simulink model "hbridge_rl_verified"  (R2026a)
settings: Solver=FixedStepDiscrete  StartTime=0  StopTime=0.42  FixedStep=1e-6
libraries: ee_lib x14, nesl_utility x8, fl_lib x4
settings Model: ModifiedByFormat=GKC3-Simulink contributors  Creator=GKC3-Simulink contributors  LastModifiedBy=GKC3-Simulink contributors
settings SolverCC: ZeroCrossControl=DisableAll
settings SimscapeCC: EditingMode=Restricted

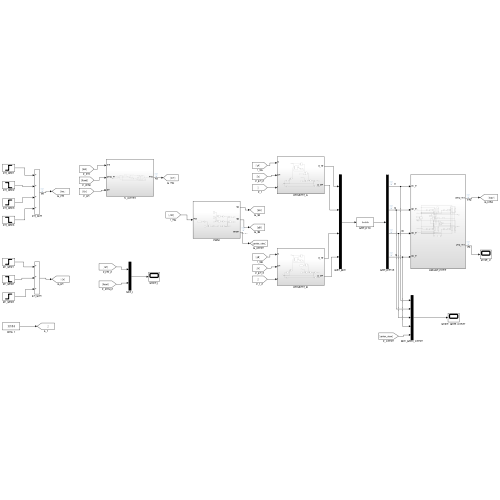
[thumbnail: Simulink's stored preview of the top-level diagram]
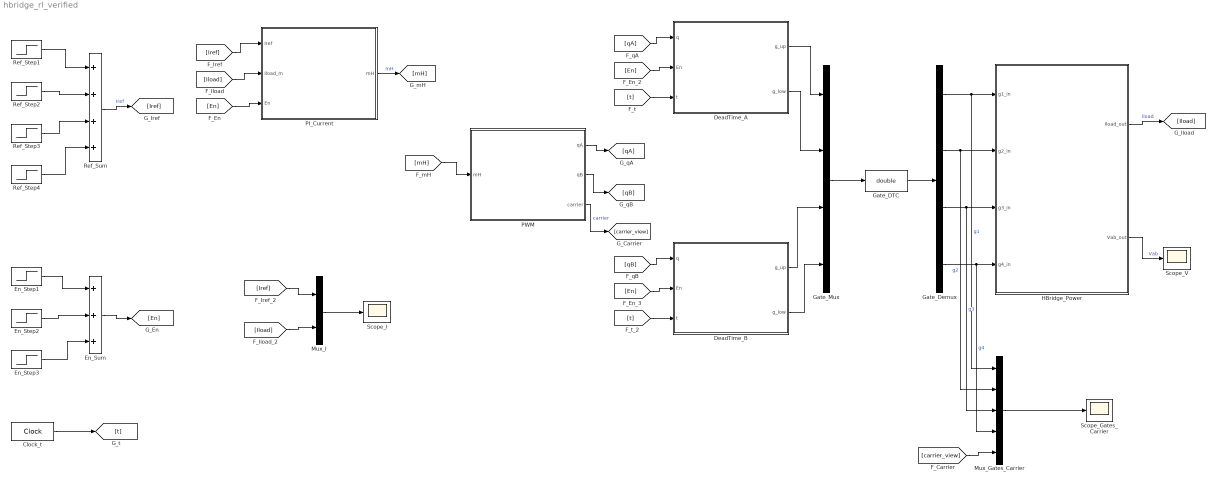
== system hbridge_rl_verified ==
  Clock_t : DigitalClock  SampleTime=1e-6
  DeadTime_A : Subsystem
  DeadTime_B : Subsystem
  En_Step1 : Step  Time=0.002  SampleTime=1e-6
  En_Step2 : Step  Time=0.30  FinalValue=-1  SampleTime=1e-6
  En_Step3 : Step  Time=0.32  SampleTime=1e-6
  En_Sum : Sum  Inputs=+++
  Gate_DTC : DataTypeConversion  OutDataTypeStr=double  SaturateOnIntegerOverflow=off  RndMeth=Floor
  Gate_Demux : Demux
  Gate_Mux : Mux
  HBridge_Power : Subsystem
  Mux_Gates_Carrier : Mux  Inputs=5
  Mux_I : Mux  Inputs=2
  PI_Current : Subsystem
  PWM : Subsystem
  Ref_Step1 : Step  Time=0.02  FinalValue=500  SampleTime=50e-6
  Ref_Step2 : Step  Time=0.12  FinalValue=-1000  SampleTime=50e-6
  Ref_Step3 : Step  Time=0.24  FinalValue=800  SampleTime=50e-6
  Ref_Step4 : Step  Time=0.36  FinalValue=-300  SampleTime=50e-6
  Ref_Sum : Sum  Inputs=++++
  Scope_Gates_Carrier : Scope
  Scope_I : Scope
  Scope_V : Scope
  wires:
  Gate_Mux/1 -> Gate_DTC/1
  DeadTime_B/2(g_low) -> Gate_Mux/4
  DeadTime_B/1(g_up) -> Gate_Mux/3
  DeadTime_A/2(g_low) -> Gate_Mux/2
  DeadTime_A/1(g_up) -> Gate_Mux/1
  [qB] -> DeadTime_B/1(q)
  [qA] -> DeadTime_A/1(q)
  [t] -> DeadTime_B/3(t)
  [t] -> DeadTime_A/3(t)
  Clock_t/1 -> [t]
  [En] -> DeadTime_B/2(En)
  [En] -> DeadTime_A/2(En)
  En_Step2/1 -> En_Sum/2
  En_Step1/1 -> En_Sum/1
  Mux_I/1 -> Scope_I/1
  [Iload] -> Mux_I/2
  [Iref] -> Mux_I/1
  Ref_Sum/1 -> [Iref]  "Iref"
  Ref_Step2/1 -> Ref_Sum/2
  Ref_Step1/1 -> Ref_Sum/1
  Ref_Step3/1 -> Ref_Sum/3
  Ref_Step4/1 -> Ref_Sum/4
  [Iref] -> PI_Current/1(Iref)
  [Iload] -> PI_Current/2(Iload_m)
  En_Step3/1 -> En_Sum/3
  En_Sum/1 -> [En]
  [En] -> PI_Current/3(En)
  PI_Current/1(mH) -> [mH]  "mH"
  Gate_DTC/1 -> Gate_Demux/1
  HBridge_Power/1(Iload_out) -> [Iload]  "Iload"
  HBridge_Power/2(Vab_out) -> Scope_V/1  "Vab"
  Mux_Gates_Carrier/1 -> Scope_Gates_Carrier/1
  Gate_Demux/1 -> Mux_Gates_Carrier/1, HBridge_Power/1(g1_in)  "g1"
  Gate_Demux/2 -> Mux_Gates_Carrier/2, HBridge_Power/2(g2_in)  "g2"
  Gate_Demux/3 -> HBridge_Power/3(g3_in), Mux_Gates_Carrier/3  "g3"
  Gate_Demux/4 -> HBridge_Power/4(g4_in), Mux_Gates_Carrier/4  "g4"
  [carrier_view] -> Mux_Gates_Carrier/5
  PWM/3(carrier) -> [carrier_view]  "carrier"
  [mH] -> PWM/1(mH)
  PWM/1(qA) -> [qA]
  PWM/2(qB) -> [qB]

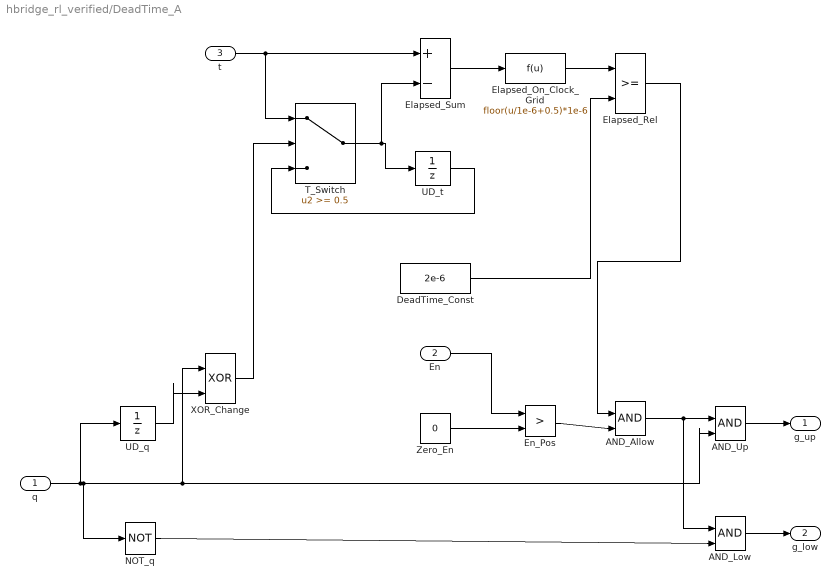
== system hbridge_rl_verified/DeadTime_A ==
  q : Inport
  En : Inport  Port=2
  t : Inport  Port=3
  AND_Allow : Logic  IconShape=distinctive  AllPortsSameDT=off  OutDataTypeStr=boolean
  AND_Low : Logic  IconShape=distinctive  AllPortsSameDT=off  OutDataTypeStr=boolean
  AND_Up : Logic  IconShape=distinctive  AllPortsSameDT=off  OutDataTypeStr=boolean
  DeadTime_Const : Constant  Value=2e-6
  Elapsed_On_Clock_Grid : Fcn  Expr=floor(u/1e-6+0.5)*1e-6
  Elapsed_Rel : RelationalOperator  OutDataTypeStr=boolean  RndMeth=Simplest  InputSameDT=off
  Elapsed_Sum : Sum  Inputs=+-
  En_Pos : RelationalOperator  Operator=>  OutDataTypeStr=boolean  RndMeth=Simplest  InputSameDT=off
  NOT_q : Logic  Operator=NOT  Inputs=1  IconShape=distinctive  AllPortsSameDT=off  OutDataTypeStr=boolean
  T_Switch : Switch  Threshold=0.5  SaturateOnIntegerOverflow=off  InputSameDT=off
  UD_q : UnitDelay  SampleTime=1e-6
  UD_t : UnitDelay  InitialCondition=-1  SampleTime=1e-6
  XOR_Change : Logic  Operator=XOR  IconShape=distinctive  AllPortsSameDT=off  OutDataTypeStr=boolean
  Zero_En : Constant  Value=0
  g_up : Outport
  g_low : Outport  Port=2
  wires:
  AND_Low/1 -> g_low/1
  AND_Up/1 -> g_up/1
  NOT_q/1 -> AND_Low/2
  AND_Allow/1 -> AND_Up/1, AND_Low/1
  En_Pos/1 -> AND_Allow/2
  Zero_En/1 -> En_Pos/2
  En/1 -> En_Pos/1
  T_Switch/1 -> UD_t/1, Elapsed_Sum/2
  UD_t/1 -> T_Switch/3
  XOR_Change/1 -> T_Switch/2
  t/1 -> Elapsed_Sum/1, T_Switch/1
  UD_q/1 -> XOR_Change/2
  q/1 -> AND_Up/2, XOR_Change/1, NOT_q/1, UD_q/1
  Elapsed_On_Clock_Grid/1 -> Elapsed_Rel/1
  Elapsed_Sum/1 -> Elapsed_On_Clock_Grid/1
  DeadTime_Const/1 -> Elapsed_Rel/2
  Elapsed_Rel/1 -> AND_Allow/1

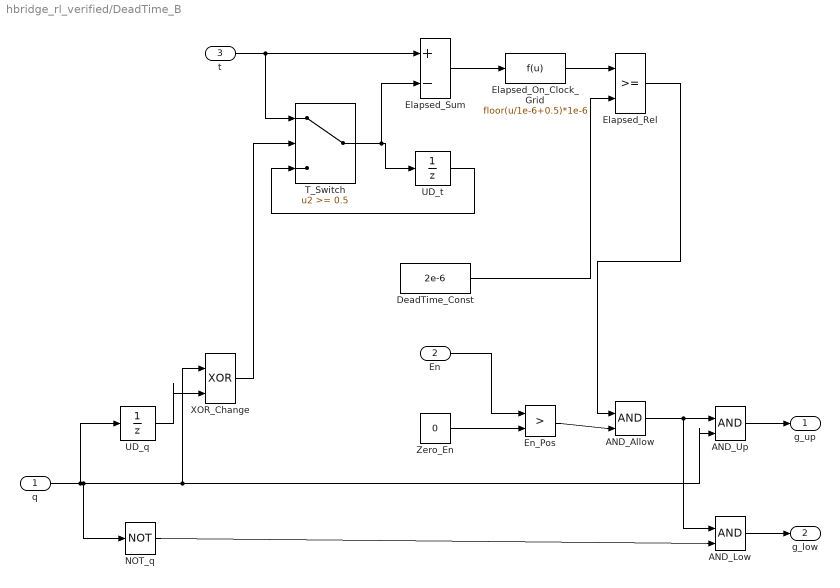
== system hbridge_rl_verified/DeadTime_B ==
  q : Inport
  En : Inport  Port=2
  t : Inport  Port=3
  AND_Allow : Logic  IconShape=distinctive  AllPortsSameDT=off  OutDataTypeStr=boolean
  AND_Low : Logic  IconShape=distinctive  AllPortsSameDT=off  OutDataTypeStr=boolean
  AND_Up : Logic  IconShape=distinctive  AllPortsSameDT=off  OutDataTypeStr=boolean
  DeadTime_Const : Constant  Value=2e-6
  Elapsed_On_Clock_Grid : Fcn  Expr=floor(u/1e-6+0.5)*1e-6
  Elapsed_Rel : RelationalOperator  OutDataTypeStr=boolean  RndMeth=Simplest  InputSameDT=off
  Elapsed_Sum : Sum  Inputs=+-
  En_Pos : RelationalOperator  Operator=>  OutDataTypeStr=boolean  RndMeth=Simplest  InputSameDT=off
  NOT_q : Logic  Operator=NOT  Inputs=1  IconShape=distinctive  AllPortsSameDT=off  OutDataTypeStr=boolean
  T_Switch : Switch  Threshold=0.5  SaturateOnIntegerOverflow=off  InputSameDT=off
  UD_q : UnitDelay  SampleTime=1e-6
  UD_t : UnitDelay  InitialCondition=-1  SampleTime=1e-6
  XOR_Change : Logic  Operator=XOR  IconShape=distinctive  AllPortsSameDT=off  OutDataTypeStr=boolean
  Zero_En : Constant  Value=0
  g_up : Outport
  g_low : Outport  Port=2
  wires:
  AND_Low/1 -> g_low/1
  AND_Up/1 -> g_up/1
  NOT_q/1 -> AND_Low/2
  AND_Allow/1 -> AND_Up/1, AND_Low/1
  En_Pos/1 -> AND_Allow/2
  Zero_En/1 -> En_Pos/2
  En/1 -> En_Pos/1
  T_Switch/1 -> UD_t/1, Elapsed_Sum/2
  UD_t/1 -> T_Switch/3
  XOR_Change/1 -> T_Switch/2
  t/1 -> Elapsed_Sum/1, T_Switch/1
  UD_q/1 -> XOR_Change/2
  q/1 -> AND_Up/2, XOR_Change/1, NOT_q/1, UD_q/1
  Elapsed_On_Clock_Grid/1 -> Elapsed_Rel/1
  Elapsed_Sum/1 -> Elapsed_On_Clock_Grid/1
  DeadTime_Const/1 -> Elapsed_Rel/2
  Elapsed_Rel/1 -> AND_Allow/1

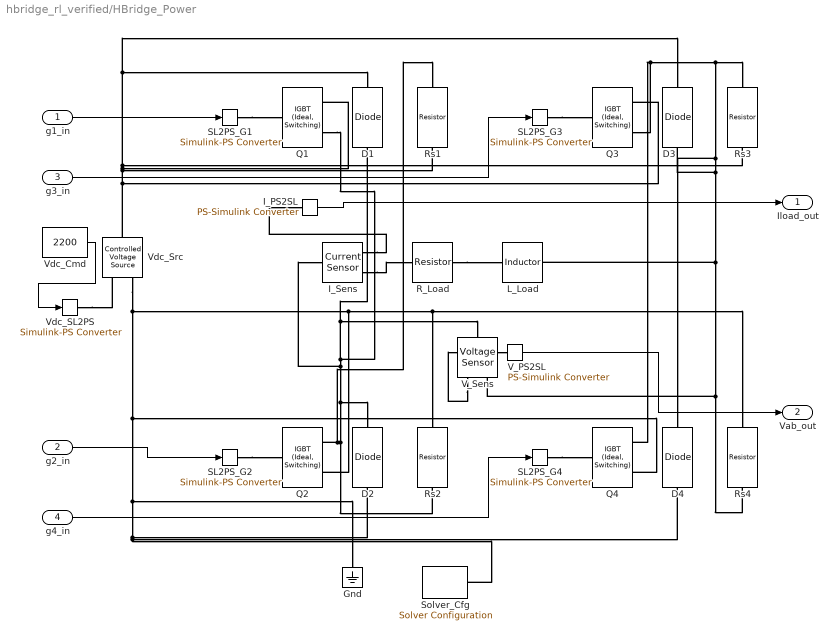
== system hbridge_rl_verified/HBridge_Power ==
  g1_in : Inport
  g2_in : Inport  Port=2
  g3_in : Inport  Port=3
  g4_in : Inport  Port=4
  D{1..4} (4 alike) : ee_lib/Semiconductors & Converters/Diode  ModelType=ee.enum.diode.modelType.pwl  TableType=ee.enum.diode.tableType.IfMat  IfMat=[.07, .12, .19, 1.75, 4.24, 7.32, 11.2; .16, .3, .72, 2.14, 5.02, 8.35, 13.12] A  VfMat=[.9, 1.15, 1.25, 1.5, 1.75, 2.17, 2.6, 2.85; .58, .68, .75, 1.1, 1.38, 1.77, 2.27, 2.7] V  TjVec=[25, 125] degC  VfVec=[.5, .7, .9, 1.3, 1.7, 2.1, 2.5] V  IfVec=[.1, .2, .5, 1, 2, 4, 7, 10] A  IrMat=[1e-06, 2e-06, 5e-06, 1e-05, 2.5e-05, 5e-05, .0001; 2e-06, 5e-06, 1e-05, 4e-05, 8e-05, .0002, .0005] A  VrMat=[10, 100, 200, 250, 300, 325, 350; 10, 70, 160, 220, 270, 300, 320] V  VrVec=[10, 20, 40, 50, 70, 80, 100] V  IrVec=[1e-06, 2e-06, 5e-06, 1e-05, 2e-05, 5e-05, .0001] A  Vf=2 V  Ron=20e-6 Ohm  Goff=1e-8 S  prmExp=ee.enum.diode.expParam.useTwo  I12=[.0137, .545] A  V12=[.6, .7] V  RS=0 Ohm  Tmeas=298.15 K  IS=1e-12 A  ec=1  I1=0.0137 A  V1=0.6 V  N_series=1  N_parallel=1  ZenerEnable=false  Rz=0.3 Ohm  BV=30 V  C_param=ee.enum.diode.capParam.fixed  CJ=0 pF  CJ0=5 pF  Vvec=[.1, 10, 100] V  Cvec=[3.5, 1, .4] pF  VJ=1 V  Mgrad=0.5  FC=0.5  Q_param=ee.enum.diode.recoveryParam.off  iRM=-7.15 A  iF=4 A  didt=-750 A/us  trr_factor=3  trr=115 ns  Qrr=150 nA*s  Vr=-600 V  Ls=150 nH  Erec=0.03 J  TT=50 ns  tau=100 ns  T_param=ee.enum.diode.temperatureParam.off  Tdevice=298.15 K  I1_T2=0.245 A  V1_T2=0.5 V  IS_T2=1.25e-7 A  Tmeas2=125 degC  XTI_param=ee.enum.diode.xtiParam.pn  XTI=3  EG_param=ee.enum.diode.egapParam.material_si  EG=1.11 eV  dBVdT=0 V/K  enable_fault_input=simscape.enum.onoff.off  i_specify=off  i_priority=None  i=0 A  i_nominal_specify=off  i_nominal_value=1  i_nominal_unit=A  v_specify=off  v_priority=None  v=0 V  v_nominal_specify=off  v_nominal_value=1  v_nominal_unit=V  v_capacitor_specify=off  v_capacitor_priority=None  v_capacitor=0 V  v_capacitor_nominal_specify=off  v_capacitor_nominal_value=1  v_capacitor_nominal_unit=V  Qj_specify=off  Qj_priority=High  Qj=0 C  Qj_nominal_specify=off  Qj_nominal_value=1  Qj_nominal_unit=C  i_diode_specify=off  i_diode_priority=None  i_diode=0 A  i_diode_nominal_specify=off  i_diode_nominal_value=1  i_diode_nominal_unit=A  v_diode_specify=off  v_diode_priority=None  v_diode=0 V  v_diode_nominal_specify=off  v_diode_nominal_value=1  v_diode_nominal_unit=V  i_capacitor_specify=off  i_capacitor_priority=None  i_capacitor=0 A  i_capacitor_nominal_specify=off  i_capacitor_nominal_value=1  i_capacitor_nominal_unit=A  fidelity_level=ee.enum.diode.fidelity.includeChargeDyn  rec_loss_model=ee.enum.diode.reverseRecoveryModelTabulateUpTo3D.fixed  ErecVal=0 J  scaleWithIandV=true  ErecMat=zeros(2, 3) J  ErecMat3D=zeros(2, 3, 2) J  TjrecVec=[298.15, 398.15] K  IfrecVec=[.1, 1, 10] A  IrecVal=10 A  VrecVal=10 V  VrecVec=[0, 100] V  tFilter=1 / 1000 / 100 s  thermal_network_parameterization=ee.enum.thermalNetworkTopology.junctionCase  Rth=[0, 10] K/W  Rth_Cauer=[1, 3, 10] K/W  Rth_Foster=[.08, .14, .22, .16] K/W  thermal_mass_parameterization=ee.enum.thermalNetwork.timeconstant  thermal_mass=[0, 1] J/K  thermal_mass_Cauer=[.1, .3, 1] J/K  thermal_mass_Foster=[.001, .005, .05, .5] J/K  thermal_time_constant=[0, 10] s  thermal_time_constant_Cauer=[1, 3, 10] s  thermal_time_constant_Foster=[7e-05, .0007, .01, .08] s  thermal_mass_initial_temperatures=[25, 25] degC  thermal_mass_initial_temperatures_Cauer=[25, 25, 25] degC  junction_thermal_mass=0.01 J/K  Tvec_initial_Foster=[25, 25, 25, 25] degC  no_thermal_network=0  junction_temperature_specify=off  junction_temperature_priority=None  junction_temperature=25 degC  junction_temperature_nominal_specify=off  junction_temperature_nominal_value=1  junction_temperature_nominal_unit=degC
  Gnd : fl_lib/Electrical/Electrical Elements/Electrical Reference
  I_PS2SL : nesl_utility/PS-Simulink Converter  PhysicalDomain=network_engine_domain  SubClassName=ps_output  LeftPortType=input  RightPortType=output  PseudoPeriodic=off  Frequencies=[]  VectorFormat=inherit  Unit=A  AffineConversion=off
  I_Sens : fl_lib/Electrical/Electrical Sensors/Current Sensor
  L_Load : ee_lib/Passive/Inductor  l=20e-3 H  enable_L_tol=ee.enum.toleranceApplication.none  L_tol=20  tol_distribution=ee.enum.toleranceDistribution.uniform  nSigma=4  r=0 Ohm  g=0 1/Ohm  enable_operating_limits=ee.enum.enable.no  operating_limit_action=ee.enum.passive.reportOpLim.warn  max_working_current=1 A  power_rating=1 W  i_L_specify=on  i_L_priority=High  i_L=0 A  i_L_nominal_specify=off  i_L_nominal_value=1  i_L_nominal_unit=A
  Q{1..4} (4 alike) : ee_lib/Semiconductors & Converters/IGBT (Ideal, Switching)  port_option=ee.enum.controlport.ps  Vf=2 V  Ron=20e-6 Ohm  Goff=1e-8 1/Ohm  Vth=0.5 V  diode_param=ee.enum.semiconductors.protectionDiode.external  diode_Vf=0.8 V  diode_Ron=0.001 Ohm  diode_Goff=1e-5 1/Ohm  diode_C=50e-9 F  diode_iRM=-235 A  diode_iF=300 A  diode_idot=-50 A/us  diode_trr_param=ee.enum.converters.diodeReverseParam.trr_factor  diode_trr_factor=3  diode_trr=15 us  diode_Qrr=1500 s*uA  ice_specify=off  ice_priority=None  ice=0 A  ice_nominal_specify=off  ice_nominal_value=1  ice_nominal_unit=A  vce_specify=off  vce_priority=None  vce=0 V  vce_nominal_specify=off  vce_nominal_value=1  vce_nominal_unit=V  vge_specify=off  vge_priority=None  vge=0 V  vge_nominal_specify=off  vge_nominal_value=1  vge_nominal_unit=V  thermal_loss_option=ee.enum.converters.thermalLossOption.constantvalues  Von_data=[0, .1, .6, .8, 1, 1.3, 1.6, 2, 2.4; 0, .1, .7, 1, 1.2, 1.5, 1.9, 2.4, 2.8] V  Tj=[298.15, 398.15] K  Iout_data=[0, .1, 1, 5, 10, 20, 40, 70, 100] A  tabulateWithVce=false  Eon_data=[0, .0024, .024, .12, .2, .48, 1.04, 2.16, 3.24; 0, .003, .03, .15, .25, .6, 1.3, 2.7, 4.05] * 1e-3 J  Eoff_data=[0, .0007, .0066, .033, .066, .17, .33, .83, 1.5; 0, .001, .01, .05, .1, .25, .5, 1.2, 2.2] * 1e-3 J  Eon_data_3D=[zeros(2, 9, 3)] J  Eoff_data_3D=[zeros(2, 9, 3)] J  Tj_loss=[298.15, 398.15] K  Iout_data_loss=[0, .1, 1, 5, 10, 20, 40, 70, 100] A  Vce_loss=[0, 150, 300] V  Eon_scalar=22.86e-3 J  Eoff_scalar=17.14e-3 J  Voff=300 V  Iout_scalar=600 A  useCurrentFromPreviousCycle=false  useVoltageFromPreviousCycle=false  diodeModelType=ee.enum.converters.diodeModelType.pwl  diodeTableType=ee.enum.diode.tableType.IfMat  diode_ReverseIVType=ee.enum.diode.diodeReverseIV.constant  diode_IfMat=[.07, .12, .19, 1.75, 4.24, 7.32, 11.2; .16, .3, .72, 2.14, 4.02, 6.35, 9.12] A  diode_VfMat=[.9, 1.15, 1.25, 1.5, 1.75, 2.17, 2.6, 2.85; .58, .68, .75, 1.1, 1.38, 1.77, 2.27, 2.7] V  diode_TjVec=[25, 125] degC  diode_VfVec=[.5, .7, .9, 1.3, 1.7, 2.1, 2.5] V  diode_IfVec=[.1, .2, .5, 1, 2, 4, 7, 10] A  diode_IrMat=[1e-06, 2e-06, 5e-06, 1e-05, 2.5e-05, 5e-05, .0001; 2e-06, 5e-06, 1e-05, 4e-05, 8e-05, .0002, .0005] A  diode_VrMat=[10, 100, 200, 250, 300, 325, 350; 10, 70, 160, 220, 270, 300, 320] V  diode_VrVec=[10, 20, 40, 50, 70, 80, 100] V  diode_IrVec=[1e-06, 2e-06, 5e-06, 1e-05, 2e-05, 5e-05, .0001] A  diode_Vr=-600 V  diode_Ls=150 nH  diode_Erec=0.03 J  diode_rec_loss_model=ee.enum.diode.reverseRecoveryModelTabulateUpTo3D.fixed  diode_ErecVal=0 J  diode_scaleWithIandV=true  diode_ErecMat=zeros(2, 3) J  diodeErecMat3D=zeros(2, 3, 2) J  diode_TjrecVec=[298.15, 398.15] K  diode_IfrecVec=[.1, 1, 10] A  diodeVrecVec=[0, 100] V  diode_IrecVal=10 A  diode_VrecVal=10 V  diode_tFilter=1 / 1000 / 100 s  separateThermalPortForDiode=false  thermal_network_parameterization=ee.enum.thermalNetworkTopology.external  Rth=[.08, .5] K/W  Rth_Cauer=[.08, .1, .5] K/W  Rth_Foster=[.08, .14, .22, .16] K/W  thermal_mass_parameterization=ee.enum.thermalNetwork.timeconstant  thermal_mass=[.01, .5] J/K  thermal_mass_Cauer=[.01, .1, .5] J/K  thermal_mass_Foster=[.001, .005, .05, .5] J/K  thermal_time_constant=[.001, .2] s  thermal_time_constant_Cauer=[.001, .1, .2] s  thermal_time_constant_Foster=[7e-05, .0007, .01, .08] s  thermal_mass_initial_temperatures=[25, 25] degC  thermal_mass_initial_temperatures_Cauer=[25, 25, 25] degC  junction_thermal_mass=0.01 J/K  Tvec_initial_Foster=[25, 25, 25, 25] degC  RthDiode=[.03, .2] K/W  RthCauerDiode=[.03, .1, .2] K/W  RthFosterDiode=[.03, .2] K/W  thermalMassDiode=[3, 25] J/K  thermalMassCauerDiode=[3, 10, 25] J/K  thermalMassFosterDiode=[33, 50] J/K  thermalTauDiode=[.1, 5] s  thermalTauCauerDiode=[.1, 1, 5] s  thermalTauFosterDiode=[1, 10] s  thermalMassInitTempDiode=[25, 25] degC  thermalMassInitTempCauerDiode=[25, 25, 25] degC  junctionthermalMassDiode=0.1 J/K  TVecInitialFosterDiode=[25, 25, 25, 25] degC  no_thermal_network=ee.enum.enable.no  IGBT_junction_temperature_specify=off  IGBT_junction_temperature_priority=None  IGBT_junction_temperature=25 degC  IGBT_junction_temperature_nominal_specify=off  IGBT_junction_temperature_nominal_value=1  IGBT_junction_temperature_nominal_unit=degC  diode_junction_temperature_specify=off  diode_junction_temperature_priority=None  diode_junction_temperature=25 degC  diode_junction_temperature_nominal_specify=off  diode_junction_temperature_nominal_value=1  diode_junction_temperature_nominal_unit=degC  Qj_specify=off  Qj_priority=None  Qj=0 W  Qj_nominal_specify=off  Qj_nominal_value=1  Qj_nominal_unit=W  accumulatedSwitchingLosses_specify=off  accumulatedSwitchingLosses_priority=None  accumulatedSwitchingLosses=0 J
  R_Load : ee_lib/Passive/Resistor  R=0.2 Ohm  enable_R_tol=ee.enum.toleranceApplication.none  R_tol=5  tol_distribution=ee.enum.toleranceDistribution.uniform  nSigma=4  enable_operating_limits=ee.enum.enable.no  operating_limit_action=ee.enum.passive.reportOpLim.warn  power_rating=1 W  max_working_voltage=100 V  noise_mode=ee.enum.sources.noise.Disabled  Tdevice=25 degC  sample_time=1e-3 s  repeatability=ee.enum.ic.repeatability.notRepeatable  user_seed=0  auto_seed=1913778160  power_derating_T1=70 degC  power_derating_T2=155 degC  operating_temperature_range_vec=[-50, 150] degC  alpha=3.93e-3 1/K  Tmeas=25 degC  thermal_mass=100 J/K  temperature_specify=off  temperature_priority=High  temperature=298.15 K  temperature_nominal_specify=off  temperature_nominal_value=1  temperature_nominal_unit=K
  Rs1 : ee_lib/Passive/Resistor  R=1e7 Ohm  enable_R_tol=ee.enum.toleranceApplication.none  R_tol=5  tol_distribution=ee.enum.toleranceDistribution.uniform  nSigma=4  enable_operating_limits=ee.enum.enable.no  operating_limit_action=ee.enum.passive.reportOpLim.warn  power_rating=1 W  max_working_voltage=100 V  noise_mode=ee.enum.sources.noise.Disabled  Tdevice=25 degC  sample_time=1e-3 s  repeatability=ee.enum.ic.repeatability.notRepeatable  user_seed=0  auto_seed=3287869569  power_derating_T1=70 degC  power_derating_T2=155 degC  operating_temperature_range_vec=[-50, 150] degC  alpha=3.93e-3 1/K  Tmeas=25 degC  thermal_mass=100 J/K  temperature_specify=off  temperature_priority=High  temperature=298.15 K  temperature_nominal_specify=off  temperature_nominal_value=1  temperature_nominal_unit=K
  Rs2 : ee_lib/Passive/Resistor  R=1e7 Ohm  enable_R_tol=ee.enum.toleranceApplication.none  R_tol=5  tol_distribution=ee.enum.toleranceDistribution.uniform  nSigma=4  enable_operating_limits=ee.enum.enable.no  operating_limit_action=ee.enum.passive.reportOpLim.warn  power_rating=1 W  max_working_voltage=100 V  noise_mode=ee.enum.sources.noise.Disabled  Tdevice=25 degC  sample_time=1e-3 s  repeatability=ee.enum.ic.repeatability.notRepeatable  user_seed=0  auto_seed=3415357569  power_derating_T1=70 degC  power_derating_T2=155 degC  operating_temperature_range_vec=[-50, 150] degC  alpha=3.93e-3 1/K  Tmeas=25 degC  thermal_mass=100 J/K  temperature_specify=off  temperature_priority=High  temperature=298.15 K  temperature_nominal_specify=off  temperature_nominal_value=1  temperature_nominal_unit=K
  Rs3 : ee_lib/Passive/Resistor  R=1e7 Ohm  enable_R_tol=ee.enum.toleranceApplication.none  R_tol=5  tol_distribution=ee.enum.toleranceDistribution.uniform  nSigma=4  enable_operating_limits=ee.enum.enable.no  operating_limit_action=ee.enum.passive.reportOpLim.warn  power_rating=1 W  max_working_voltage=100 V  noise_mode=ee.enum.sources.noise.Disabled  Tdevice=25 degC  sample_time=1e-3 s  repeatability=ee.enum.ic.repeatability.notRepeatable  user_seed=0  auto_seed=802611725  power_derating_T1=70 degC  power_derating_T2=155 degC  operating_temperature_range_vec=[-50, 150] degC  alpha=3.93e-3 1/K  Tmeas=25 degC  thermal_mass=100 J/K  temperature_specify=off  temperature_priority=High  temperature=298.15 K  temperature_nominal_specify=off  temperature_nominal_value=1  temperature_nominal_unit=K
  Rs4 : ee_lib/Passive/Resistor  R=1e7 Ohm  enable_R_tol=ee.enum.toleranceApplication.none  R_tol=5  tol_distribution=ee.enum.toleranceDistribution.uniform  nSigma=4  enable_operating_limits=ee.enum.enable.no  operating_limit_action=ee.enum.passive.reportOpLim.warn  power_rating=1 W  max_working_voltage=100 V  noise_mode=ee.enum.sources.noise.Disabled  Tdevice=25 degC  sample_time=1e-3 s  repeatability=ee.enum.ic.repeatability.notRepeatable  user_seed=0  auto_seed=2103522063  power_derating_T1=70 degC  power_derating_T2=155 degC  operating_temperature_range_vec=[-50, 150] degC  alpha=3.93e-3 1/K  Tmeas=25 degC  thermal_mass=100 J/K  temperature_specify=off  temperature_priority=High  temperature=298.15 K  temperature_nominal_specify=off  temperature_nominal_value=1  temperature_nominal_unit=K
  SL2PS_G{1..4} (4 alike) : nesl_utility/Simulink-PS Converter  PhysicalDomain=network_engine_domain  SubClassName=ps_input  LeftPortType=input  RightPortType=output  PseudoPeriodic=off  Frequencies=[]  NoiseDistribution=none  NoiseParameters=[]  Unit=V  AffineConversion=off  FilteringAndDerivatives=zero  SimscapeFilterOrder=1  InputFilterTimeConstant=0.001  UdotUserProvided=0
  Solver_Cfg : nesl_utility/Solver Configuration  PhysicalDomain=network_engine_domain  SubClassName=solver  LeftPortType=input  RightPortType=generic  Tones=[]  Harmonics=[]  SimulateNoise=off  Profile=off  UseLocalSampling=off  EnableSwitchedLinearOptims=on  FrequencyDomain=off  UseCCode=off  RelTol=0.001  AbsTol=0.001  MinStep=1e-09  ToWorkspace=off  RevertToSquareIcSolve=off  NumHomotopyIterations=100  PhasorMode=off  PhasorModeNumHarmonics=1  ConsistencySolver=NEWTON_XTOL_AFTER_FTOL  CanonicalOrdering=CANONICAL  OptimizeIntermediates=OPTIMIZED  IndexReductionMethod=DerivativeReplacement  DoDC=off  ResidualTolerance=1e-09  ConsistencyTolSource=GLOBAL  ConsistencyAbsTol=0.001  ConsistencyRelTol=0.001  ConsistencyTolFactor=0.001  UseLocalSolver=on  LocalSolverChoice=NE_BACKWARD_EULER_ADVANCER  ResolveIndetEquations=on  FunctionEvalNumThread=1  LocalSolverSampleTime=1e-6  DoFixedCost=on  MaxNonlinIter=3  MaxModeIter=2  ComputeImpulses=off  ImpulseIterations=2  LinearAlgebra=auto  LinearAlgebraNumThread=0  EquationFormulation=NE_TIME_EF  DelaysMemoryBudget=1024  AutomaticFiltering=on  FilteringTimeConstant=0.001  PartitionStorageMethod=AS_NEEDED  PartitionMemoryBudget=1024  PartitionMethod=ROBUST  MultibodyUseLocalSolver=off  MultibodyLocalSolverChoice=ODE1  MultibodyLocalSolverSampleTime=0.001
  V_PS2SL : nesl_utility/PS-Simulink Converter  PhysicalDomain=network_engine_domain  SubClassName=ps_output  LeftPortType=input  RightPortType=output  PseudoPeriodic=off  Frequencies=[]  VectorFormat=inherit  Unit=V  AffineConversion=off
  V_Sens : fl_lib/Electrical/Electrical Sensors/Voltage Sensor
  Vdc_Cmd : Constant  Value=2200
  Vdc_SL2PS : nesl_utility/Simulink-PS Converter  PhysicalDomain=network_engine_domain  SubClassName=ps_input  LeftPortType=input  RightPortType=output  PseudoPeriodic=off  Frequencies=[]  NoiseDistribution=none  NoiseParameters=[]  Unit=V  AffineConversion=off  FilteringAndDerivatives=zero  SimscapeFilterOrder=1  InputFilterTimeConstant=0.001  UdotUserProvided=0
  Vdc_Src : fl_lib/Electrical/Electrical Sources/Controlled Voltage Source
  Iload_out : Outport
  Vab_out : Outport  Port=2
  wires:
  Vdc_Cmd/1 -> Vdc_SL2PS/1
  V_PS2SL/1 -> Vab_out/1
  I_PS2SL/1 -> Iload_out/1
  g4_in/1 -> SL2PS_G4/1
  g3_in/1 -> SL2PS_G3/1
  g2_in/1 -> SL2PS_G2/1
  g1_in/1 -> SL2PS_G1/1
  connections:
  V_Sens/RConn1 -- V_PS2SL/LConn1
  I_Sens/RConn1 -- I_PS2SL/LConn1
  SL2PS_G4/RConn1 -- Q4/LConn1
  SL2PS_G3/RConn1 -- Q3/LConn1
  SL2PS_G2/RConn1 -- Q2/LConn1
  SL2PS_G1/RConn1 -- Q1/LConn1
  Vdc_SL2PS/RConn1 -- Vdc_Src/RConn1
  R_Load/RConn1 -- L_Load/LConn1
  I_Sens/RConn2 -- R_Load/LConn1
  Q4/RConn1 -- V_Sens/RConn2 -- Rs4/LConn1 -- L_Load/RConn1 -- D3/LConn1 -- D4/RConn1 -- Rs3/RConn1 -- Q3/RConn2
  V_Sens/LConn1 -- Q2/RConn1 -- Rs1/RConn1 -- Rs2/LConn1 -- D2/RConn1 -- I_Sens/LConn1 -- Q1/RConn2 -- D1/LConn1
  Solver_Cfg/RConn1 -- Vdc_Src/RConn2 -- Rs4/RConn1 -- Rs2/RConn1 -- Q2/RConn2 -- Q4/RConn2 -- Gnd/LConn1 -- D2/LConn1 -- D4/LConn1
  Q1/RConn1 -- D1/RConn1 -- D3/RConn1 -- Rs3/LConn1 -- Vdc_Src/LConn1 -- Q3/RConn1 -- Rs1/LConn1

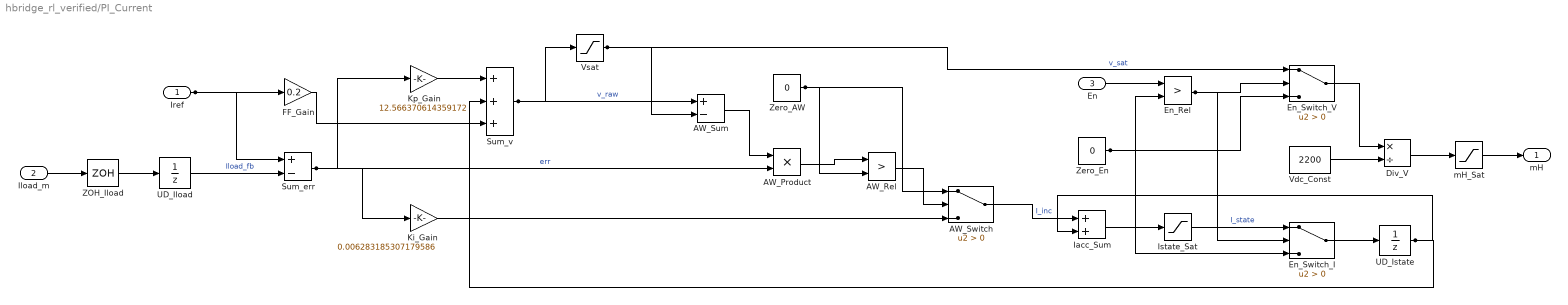
== system hbridge_rl_verified/PI_Current ==
  Iref : Inport
  Iload_m : Inport  Port=2
  En : Inport  Port=3
  AW_Product : Product
  AW_Rel : RelationalOperator  Operator=>  OutDataTypeStr=boolean  RndMeth=Simplest  InputSameDT=off
  AW_Sum : Sum  Inputs=+-
  AW_Switch : Switch  Criteria=u2 > Threshold  SaturateOnIntegerOverflow=off  InputSameDT=off
  Div_V : Product  Inputs=*/
  En_Rel : RelationalOperator  Operator=>  OutDataTypeStr=boolean  RndMeth=Simplest  InputSameDT=off
  En_Switch_I : Switch  Criteria=u2 > Threshold  SaturateOnIntegerOverflow=off  InputSameDT=off
  En_Switch_V : Switch  Criteria=u2 > Threshold  SaturateOnIntegerOverflow=off  InputSameDT=off
  FF_Gain : Gain  Gain=0.2
  Iacc_Sum : Sum
  Istate_Sat : Saturate  UpperLimit=400  LowerLimit=-400
  Ki_Gain : Gain  Gain=0.006283185307179586
  Kp_Gain : Gain  Gain=12.566370614359172
  Sum_err : Sum  Inputs=+-
  Sum_v : Sum  Inputs=+++
  UD_Iload : UnitDelay  SampleTime=50e-6
  UD_Istate : UnitDelay  SampleTime=50e-6
  Vdc_Const : Constant  Value=2200
  Vsat : Saturate  UpperLimit=400  LowerLimit=-400
  ZOH_Iload : ZeroOrderHold  SampleTime=50e-6
  Zero_AW : Constant  Value=0
  Zero_En : Constant  Value=0
  mH_Sat : Saturate  UpperLimit=0.95  LowerLimit=-0.95
  mH : Outport
  wires:
  ZOH_Iload/1 -> UD_Iload/1
  UD_Iload/1 -> Sum_err/2  "Iload_fb"
  Sum_err/1 -> Kp_Gain/1, AW_Product/2, Ki_Gain/1  "err"
  Kp_Gain/1 -> Sum_v/1
  Ki_Gain/1 -> AW_Switch/3
  Sum_v/1 -> Vsat/1, AW_Sum/1  "v_raw"
  Vsat/1 -> En_Switch_V/1, AW_Sum/2  "v_sat"
  AW_Sum/1 -> AW_Product/1
  Zero_AW/1 -> AW_Rel/2, AW_Switch/1
  AW_Product/1 -> AW_Rel/1
  AW_Rel/1 -> AW_Switch/2
  AW_Switch/1 -> Iacc_Sum/1  "I_inc"
  UD_Istate/1 -> Iacc_Sum/2, Sum_v/2
  Iacc_Sum/1 -> Istate_Sat/1
  Istate_Sat/1 -> En_Switch_I/1  "I_state"
  Zero_En/1 -> En_Switch_I/3, En_Switch_V/3, En_Rel/2
  En_Rel/1 -> En_Switch_V/2, En_Switch_I/2
  En_Switch_I/1 -> UD_Istate/1
  FF_Gain/1 -> Sum_v/3
  En_Switch_V/1 -> Div_V/1
  Vdc_Const/1 -> Div_V/2
  Div_V/1 -> mH_Sat/1
  mH_Sat/1 -> mH/1
  Iload_m/1 -> ZOH_Iload/1
  Iref/1 -> Sum_err/1, FF_Gain/1
  En/1 -> En_Rel/1

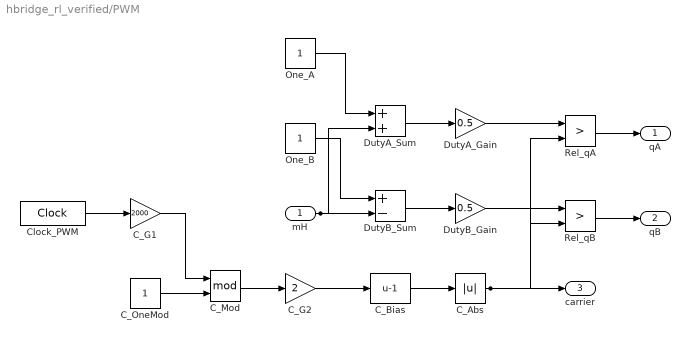
== system hbridge_rl_verified/PWM ==
  mH : Inport
  C_Abs : Abs  SaturateOnIntegerOverflow=off
  C_Bias : Bias  Bias=-1  SaturateOnIntegerOverflow=off
  C_G1 : Gain  Gain=2000
  C_G2 : Gain  Gain=2
  C_Mod : Math  Operator=mod  AlgorithmType=Exact
  C_OneMod : Constant
  Clock_PWM : DigitalClock  SampleTime=1e-6
  DutyA_Gain : Gain  Gain=0.5
  DutyA_Sum : Sum
  DutyB_Gain : Gain  Gain=0.5
  DutyB_Sum : Sum  Inputs=+-
  One_A : Constant
  One_B : Constant
  Rel_qA : RelationalOperator  Operator=>  OutDataTypeStr=boolean  RndMeth=Simplest  InputSameDT=off
  Rel_qB : RelationalOperator  Operator=>  OutDataTypeStr=boolean  RndMeth=Simplest  InputSameDT=off
  qA : Outport
  qB : Outport  Port=2
  carrier : Outport  Port=3
  wires:
  mH/1 -> DutyA_Sum/2, DutyB_Sum/2
  Rel_qB/1 -> qB/1
  Rel_qA/1 -> qA/1
  DutyB_Gain/1 -> Rel_qB/1
  C_Abs/1 -> Rel_qA/2, Rel_qB/2, carrier/1
  DutyA_Gain/1 -> Rel_qA/1
  DutyB_Sum/1 -> DutyB_Gain/1
  One_B/1 -> DutyB_Sum/1
  DutyA_Sum/1 -> DutyA_Gain/1
  One_A/1 -> DutyA_Sum/1
  C_Bias/1 -> C_Abs/1
  C_G2/1 -> C_Bias/1
  C_Mod/1 -> C_G2/1
  C_G1/1 -> C_Mod/1
  Clock_PWM/1 -> C_G1/1
  C_OneMod/1 -> C_Mod/2
